simulink model "SimulinkForSystemDesign"  (R2026a)
settings: Solver=VariableStepAuto
libraries: cstblocks_lti x2
settings Model: Creator=ms110  LastModifiedBy=ms110

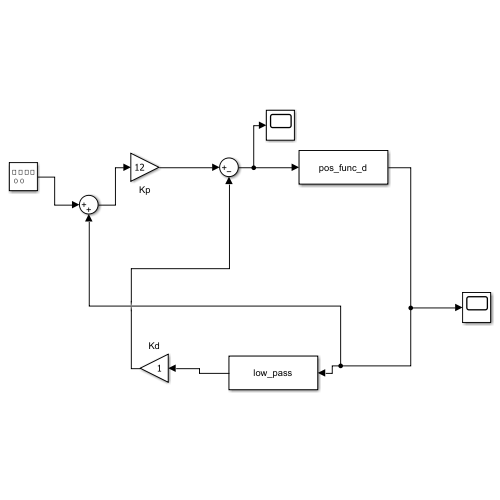
[thumbnail: Simulink's stored preview of the top-level diagram]
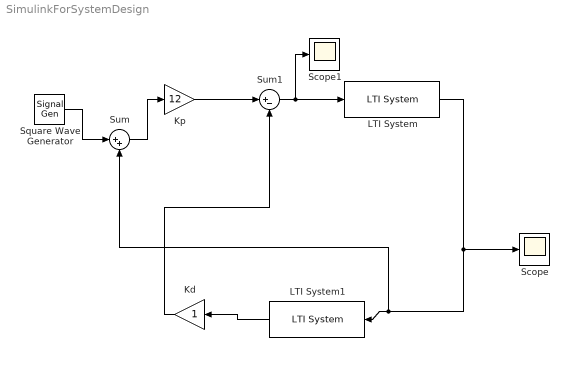
== system SimulinkForSystemDesign ==
  Kd : Gain
  Kp : Gain  Gain=12
  LTI System : cstblocks_lti/LTI System  sys=pos_func_d  IC=[]  PadeOrder=0
      settings: LibrarySourceBlock=cstblocks/LTI System
  LTI System1 : cstblocks_lti/LTI System  sys=low_pass  IC=[]  PadeOrder=0
      settings: LibrarySourceBlock=cstblocks/LTI System
  Scope : Scope
  Scope1 : Scope
  Square Wave Generator : SignalGenerator  WaveForm=square  Units=rad/sec
  Sum : Sum  Inputs=|++
  Sum1 : Sum  Inputs=|+-
  wires:
  Kp/1 -> Sum1/1
  LTI System/1 -> Scope/1, Sum/2, LTI System1/1
  LTI System1/1 -> Kd/1
  Kd/1 -> Sum1/2
  Sum1/1 -> Scope1/1, LTI System/1
  Sum/1 -> Kp/1
  Square Wave Generator/1 -> Sum/1
